simulink model "simulink_motor"  (R2025b)
settings: Solver=FixedStepAuto  StartTime=0.0  StopTime=0.5  FixedStep=0.005  RelTol=1e-3  EnableMultiTasking=on
libraries: arduinolib x2, arduinosensorlib x1
settings Model: SimulationMode=external  ExtModeTrigDuration=2  Creator=Kleiton  LastModifiedBy=Kleiton
settings SolverCC: AutoInsertRateTranBlk=on
settings OptimizationCC: EnhancedBackFolding=on  PassReuseOutputArgsAs=Individual arguments  ZeroExternalMemoryAtStartup=off  ZeroInternalMemoryAtStartup=off  MaxStackSize=64  OptimizeBlockOrder=speed  DifferentSizesBufferReuse=on  OptimizationCustomize=off  EfficientTunableParamExpr=on
settings DebuggingCC: ParameterTunabilityLossMsg=error
settings HardwareCC: ProdBitPerInt=16.0  ProdBitPerPointer=16.0  ProdBitPerSizeT=16.0  ProdBitPerPtrDiffT=16.0  ProdLargestAtomicFloat=None  ProdWordSize=8.0  ProdHWDeviceType=Atmel->AVR
settings SFSimCC: MATLABDynamicMemAlloc=off
settings RTWCC: SystemTargetFile=ert.tlc  HardwareBoard=Arduino Uno  TemplateMakefile=ert_default_tmf  Toolchain=Arduino AVR  BuildConfiguration=Faster Runs  Description=Embedded Coder
settings CodeAppCC: ForceParamTrailComments=on  IgnoreCustomStorageClasses=off  OperatorAnnotations=on  SimulinkDataObjDesc=on  SFDataObjDesc=on  InsertBlockDesc=on
settings ERTTargetCC: ExtModeTransport=3.0  ExtModeStaticAlloc=on  ExtModeAutomaticAllocSize=off  ExtModeStaticAllocSize=250.0  ExtModeMexFile=ext_xcp  ExtModeIntrfLevel=Level2 - Open  InlinedParameterPlacement=Hierarchical  SupportContinuousTime=on  SupportVariableSizeSignals=on

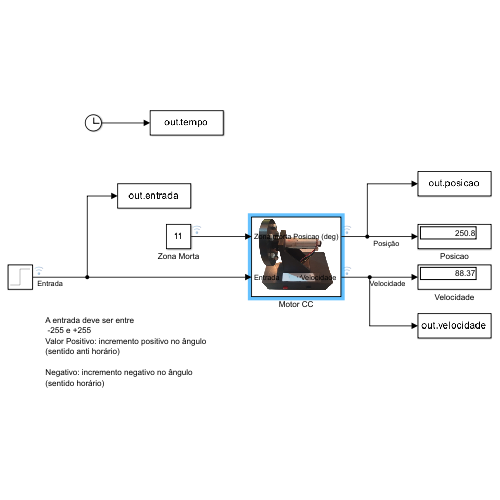
[thumbnail: Simulink's stored preview of the top-level diagram]
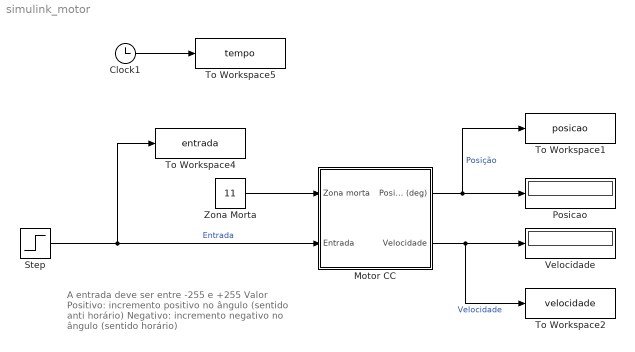
== system simulink_motor ==
  note: A entrada deve ser entre
      |  -255 e +255
      | Valor Positivo: incremento positivo no ângulo
      | (sentido anti horário)
      |
      | Negativo: incremento negativo no ângulo
      | (sentido horário)
  Clock1 : Clock
  Motor CC : Subsystem
      mask Display: image('motor_cc.png');
  Posicao : Display
  Step : Step  Time=0  After=100  SampleTime=0
  To Workspace1 : ToWorkspace  VariableName=posicao  SampleTime=-1
      settings: Save2DSignal=2-D array (concatenate along first dimension)
  To Workspace2 : ToWorkspace  VariableName=velocidade  SampleTime=-1
      settings: Save2DSignal=2-D array (concatenate along first dimension)
  To Workspace4 : ToWorkspace  VariableName=entrada  SampleTime=-1
      settings: Save2DSignal=2-D array (concatenate along first dimension)
  To Workspace5 : ToWorkspace  VariableName=tempo  SampleTime=-1
      settings: Save2DSignal=2-D array (concatenate along first dimension)
  Velocidade : Display
  Zona Morta : Constant  Value=11
  wires:
  Motor CC/1(Posicao (deg)) -> Posicao/1, To Workspace1/1  "Posição"
  Clock1/1 -> To Workspace5/1
  Zona Morta/1 -> Motor CC/1(Zona morta)
  Motor CC/2("Velocidade ") -> To Workspace2/1, Velocidade/1  "Velocidade"
  Step/1 -> To Workspace4/1, Motor CC/2(Entrada)  "Entrada"

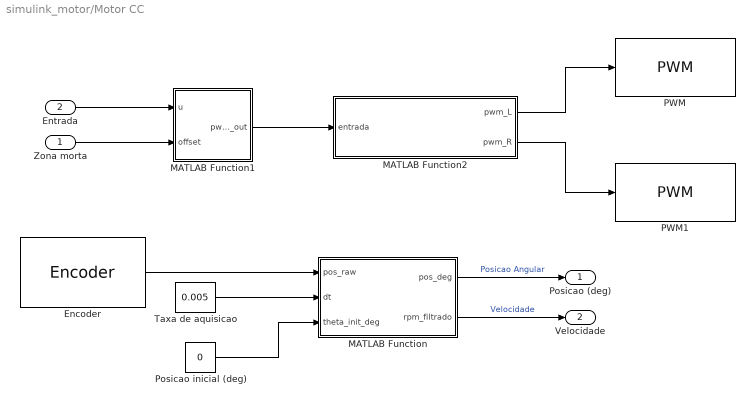
== system simulink_motor/Motor CC ==
  Zona morta : Inport
  Entrada : Inport  Port=2
  Encoder : arduinosensorlib/Encoder  InputA=2  InputB=3  Mode=No reset  SampleTime=0.005
  MATLAB Function : MATLAB Function  TreatAsAtomicUnit=on
  MATLAB Function1 : MATLAB Function  TreatAsAtomicUnit=on
  MATLAB Function2 : MATLAB Function  TreatAsAtomicUnit=on
  PWM : arduinolib/PWM  pinNumber=9  frequencyType=Specify  desiredFrequency=3921.16  achievableFrequency=3921.5686
  PWM1 : arduinolib/PWM  pinNumber=10  frequencyType=Specify  desiredFrequency=3921.16  achievableFrequency=3921.5686
  Posicao inicial (deg) : Constant  Value=0
  Taxa de aquisicao : Constant  Value=0.005  VectorParams1D=off
  Posicao (deg) : Outport
  "Velocidade " : Outport  Port=2
  wires:
  Zona morta/1 -> MATLAB Function1/2(offset)
  MATLAB Function/1(pos_deg) -> Posicao (deg)/1  "Posicao Angular"
  Taxa de aquisicao/1 -> MATLAB Function/2(dt)
  Posicao inicial (deg)/1 -> MATLAB Function/3(theta_init_deg)
  Encoder/1 -> MATLAB Function/1(pos_raw)
  MATLAB Function1/1(pwm_out) -> MATLAB Function2/1(entrada)
  MATLAB Function2/1(pwm_L) -> PWM/1
  MATLAB Function2/2(pwm_R) -> PWM1/1
  Entrada/1 -> MATLAB Function1/1(u)
  MATLAB Function/2(rpm_filtrado) -> "Velocidade "/1  "Velocidade"

== matlab function simulink_motor/Motor CC/MATLAB Function2 ==
  data: entrada input; pwm_L output; pwm_R output
function [pwm_L, pwm_R] = controlar_motor(entrada)
% CONTROLAR_MOTOR Divisão de sinal para Ponte H (BTS7960)
% Entrada: entrada (-255 a 255)
% Saídas:
%   pwm_L -> LPWM - Sentido Anti-horário
%   pwm_9  -> RPWM - Sentido Horário

    if entrada > 0
        % PWM Positivo: Ativa Pino 10, Zera Pino 9
        pwm_L = entrada;
        pwm_R  = 0;
        
    elseif entrada < 0
        % PWM Negativo: Converte para positivo, Ativa Pino 9, Zera Pino 10
        pwm_L = 0;
        pwm_R  = abs(entrada);
        
    else
        % PWM Igual a Zero: Freio (Ambos zerados)
        pwm_L = 0;
        pwm_R  = 0;
    end
end

== matlab function simulink_motor/Motor CC/MATLAB Function ==
  data: pos_raw input; pos_deg output; dt input; rpm_filtrado output; theta_init_deg input
function [pos_deg, rpm_filtrado] = fcn(pos_raw, dt, theta_init_deg)
    % Converte entradas para double para evitar estouro/incompatibilidade de tipos
    pos = double(pos_raw);
    theta_init = double(theta_init_deg); % Ângulo inicial em graus
    
    % Variáveis persistentes para histórico entre amostras
    persistent offset pos_anterior rpm_anterior is_initialized;
    
    % 1. Parâmetros do Motor GA25-370 (Redução 1:46.85)
    ppr_motor = 11;                          % Pulsos nativos do disco magnético
    cpr_simulink = ppr_motor * 4;            % Quadratura 4x do Simulink (44 contagens/volta)
    reducao_caixa = 46.85;                   % Redução mecânica interna da caixa
    
    cpr_saida = cpr_simulink * reducao_caixa; % 2061.4 contagens por volta completa na saída
    
    % 2. Inicialização na primeira execução (t = 0)
    if isempty(is_initialized)
        offset = pos;
        pos_anterior = theta_init; % Posição inicial do histórico em graus
        rpm_anterior = 0;          % RPM filtrado do ciclo anterior
        is_initialized = true;
    end
    
    % 3. Posição Angular em Graus (Saída do Motor + Offset Inicial)
    pulsos_relativos = pos - offset;
    pos_deg = (pulsos_relativos * (360 / cpr_saida)) + theta_init;
    
    % 4. Velocidade Instantânea em RPM (Derivada Discreta baseada em Graus)
    if dt > 0
        d_deg = pos_deg - pos_anterior;
        % Conversão: (deg / dt) * (1 volta / 360 deg) * (60 s / 1 min) = RPM
        rpm_raw = (d_deg / dt) * (60 / 360);
    else
        rpm_raw = 0;
    end
    
    % 5. Filtro Passa-Baixas Exponencial (IIR de 1ª Ordem)
    fc = 5.0; % Frequência de corte em Hz
    tau = 1 / (2 * pi * fc);
    alpha = dt / (tau + dt); % Fator de suavização proporcional a dt
    
    rpm_filtrado = alpha * rpm_raw + (1 - alpha) * rpm_anterior;
    
    % 6. Atualiza as variáveis para a próxima amostragem
    pos_anterior = pos_deg;
    rpm_anterior = rpm_filtrado;
end

== matlab function simulink_motor/Motor CC/MATLAB Function1 ==
  data: u input; pwm_out output; offset input
function pwm_out = compensador_avancado(u, offset)
    limiar = 0; % Margem para ignorar ruído em torno de zero

    if u > limiar
        pwm_out = u + offset;
    elseif u < -limiar
        pwm_out = u - offset;
    else
        pwm_out = 0; % Não ativa o motor para ruídos residuais
    end

    % Saturação do sinal de saída para o limite do PWM (-255 a 255)
    pwm_out = min(max(pwm_out, -255), 255);
end
